simulink model "sf_gearbox"  (R2025b)
settings: Solver=FixedStepDiscrete  StartTime=0.0  StopTime=10  FixedStep=0.01  RelTol=1e-3
libraries: simulink x1
settings Model: Creator=jbjtfy  LastModifiedBy=jbjtfy

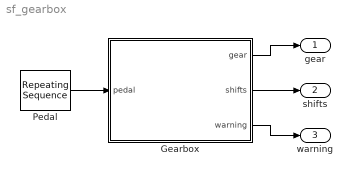
== system sf_gearbox ==
  Gearbox : Stateflow chart  TreatAsAtomicUnit=on
  Pedal : simulink/Sources/Repeating Sequence  rep_seq_t=[0 1 3 5 6 8 10]  rep_seq_y=[0 0.8 0.8 0.2 0 0.6 0]
  gear : Outport
  shifts : Outport  Port=2
  warning : Outport  Port=3
  wires:
  Gearbox/3(warning) -> warning/1
  Gearbox/2(shifts) -> shifts/1
  Gearbox/1(gear) -> gear/1
  Pedal/1 -> Gearbox/1(pedal)

== stateflow chart sf_gearbox/Gearbox ==
  settings: updateMethod=DISCRETE  sampleTime=0.01
  state Gear [parallel]
    settings: executionOrder=1
    state Driving
      exit: shifts = shifts + 1;
      state Low
        entry: gear = 1;
      state High
        entry: gear = 2;
      (default) -> Low
      Low -> High : after(1, sec)[pedal > 0.5]
    state Parked
      entry: gear = 0;
    (default) -> Parked : {gear = 0; shifts = 0;}
    High -> Low : [pedal < 0.3]
    Parked -> Driving : [pedal > 0.1]
    (junction 16) -> Parked
    Driving -> (junction 16) : [pedal < 0.05]
  state Monitor [parallel]
    settings: executionOrder=2
    state Ok
      entry: warning = 0;
    state Busy
      entry: warning = 1;
    (default) -> Ok : {warning = 0;}
    Ok -> Busy : [shifts >= 2]
  Busy -> Ok : after(2, sec)
  data: pedal input double; gear output double =0; shifts output double =0; warning output double =0
